simulink library "vlm_wing_lib"  (R2018b)
settings: Solver=VariableStepAuto  StartTime=0.0  StopTime=10.0  RelTol=1e-3
values from neighbouring files (symbols this model uses):
  wing = wingSetAeroState( wing, [0;0;0] )    [wingGet3dPolar.m]
undefined symbols (not defined in the file or in its folder): wing_struct, wing_struct_state, wing_struct_state_bus
libraries: $bdroot x6
settings Model: Creator=Ybeyer  LastModifiedBy=yannic
settings SFSimCC: SimUseLocalCustomCode=off
settings RTWCC: RTWUseLocalCustomCode=off
settings CodeAppCC: StateflowObjectComments=on

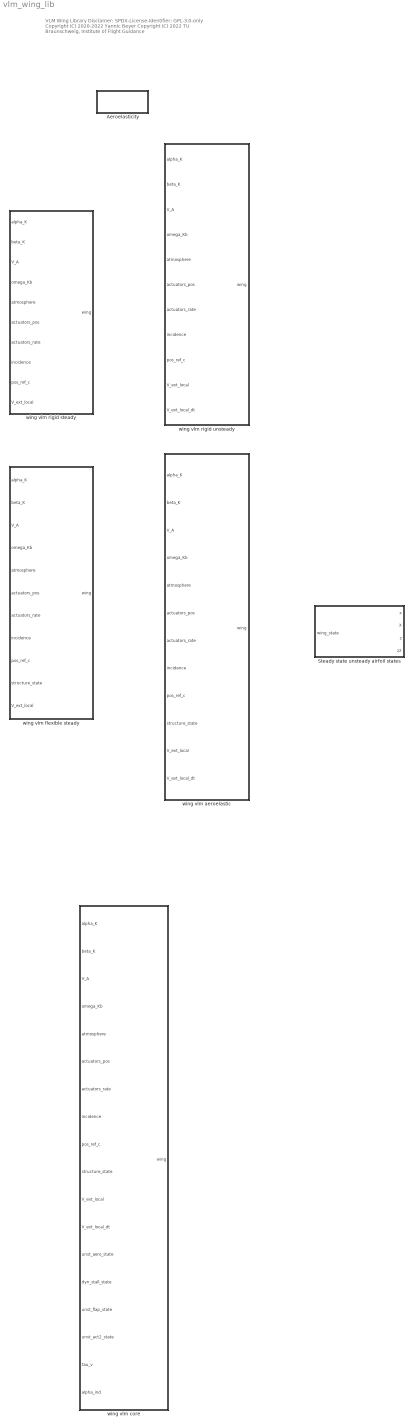
== system vlm_wing_lib ==
  note: VLM Wing Library
      |
      | Disclamer:
      | SPDX-License-Identifier: GPL-3.0-only
      |
      | Copyright (C) 2020-2022 Yannic Beyer
      | Copyright (C) 2022 TU Braunschweig, Institute of Flight Guidance
  Aeroelasticity : Subsystem
      settings: OpenFcn=aeroelasticity_lib
  Steady state unsteady airfoil states : Subsystem  mask{wing_airfoil=wing.airfoil, wing_config=wing.config}
      mask prompts: wing_airfoil "wing airfoil struct"; wing_config "wing config struct"
      mask DialogControl DescGroupVar Prompt: Compute steady state unsteady airfoil states
  wing vlm aeroelastic : Subsystem  mask{wing_struct=wing_struct, wing_state_bus=wing_struct_state, unst_aero_state_init=0, dyn_stall_state_init=0, unst_flap_state_init=0, unst_act2_state_init=0, tau_v_init=0, alpha_ind_init=0}
      mask prompts: wing_struct "Wing struct"; wing_state_bus "Wing state bus"; unst_aero_state_init "initial unst_aero_state"; dyn_stall_state_init "initial dyn_stall_state"; unst_flap_state_init "initial unst_flap_state"; unst_act2_state_init "initial unst_act2_state"; tau_v_init "initial tau_v"; alpha_ind_init "initial alpha_ind"
      mask Help: web('https://git.iff.ing.tu-bs.de/dev/flugmechanik/fdm/ladac/-/blob/feature/wing_improve_organization/aerodynamics/vlm_wing/README.md','-browser')
      mask DialogControl DescGroupVar Prompt: Wing with nonlinear vortex lattice method (aeroelastic)
      mask DialogControl DescTextVar Prompt: This block computes the aerodynamics of a wing based on the nonlinear vortex lattice method. It considers a flexible structure and unsteady aerodynamics.
      mask DialogControl Control12 Prompt: The inputs and outputs are described in the README:
      mask DialogControl Control5 Prompt: README
      mask DialogControl Control5 Callback: web('https://github.com/iff-gsc/LADAC/blob/main/aerodynamics/vlm_wing/README.md','-browser')
      mask DialogControl Control2 Prompt: To initialize a wing struct, please use the function wingCreate.
      mask DialogControl Control3 Prompt: The wing state bus can then be created by running wing_state_bus = struct2bus_(wing.state)
      mask DialogControl Container3 Prompt: Initial conditions
  wing vlm core : Subsystem  mask{wing_struct=wing_struct, wing_state_bus=wing_struct_state}
      mask prompts: wing_struct "Wing struct"; wing_state_bus "Wing state bus"
      mask Help: web('https://git.iff.ing.tu-bs.de/dev/flugmechanik/fdm/ladac/-/blob/feature/wing_improve_organization/aerodynamics/vlm_wing/README.md','-browser')
      mask DialogControl DescGroupVar Prompt: Wing with nonlinear vortex lattice method (aeroelastic)
      mask DialogControl DescTextVar Prompt: This block computes the aerodynamics of a wing based on the nonlinear vortex lattice method. It considers a flexible structure and unsteady aerodynamics.
      mask DialogControl Control12 Prompt: The inputs and outputs are described in the README:
      mask DialogControl Control5 Prompt: README
      mask DialogControl Control5 Callback: web('https://github.com/iff-gsc/LADAC/blob/main/aerodynamics/vlm_wing/README.md','-browser')
      mask DialogControl Control2 Prompt: To initialize a wing struct, please use the function wingCreate.
      mask DialogControl Control3 Prompt: The wing state bus can then be created by running wing_state_bus = struct2bus_(wing.state)
  wing vlm flexible steady : Subsystem  mask{wing_struct=wing_struct, wing_state_bus=wing_struct_state_bus, alpha_ind_init=0}
      mask prompts: wing_struct "Wing struct"; wing_state_bus "Wing state bus"; alpha_ind_init "initial alpha_ind"
      mask Help: web('https://git.iff.ing.tu-bs.de/dev/flugmechanik/fdm/ladac/-/blob/feature/wing_improve_organization/aerodynamics/vlm_wing/README.md','-browser')
      mask DialogControl DescGroupVar Prompt: Wing with nonlinear vortex lattice method (flexible steady)
      mask DialogControl DescTextVar Prompt: This block computes the aerodynamics of a wing based on the nonlinear vortex lattice method. It considers a flexible structure and steady aerodynamics.
      mask DialogControl Control2 Prompt: The inputs and outputs are described in the README:
      mask DialogControl Control5 Prompt: README
      mask DialogControl Control5 Callback: web('https://github.com/iff-gsc/LADAC/blob/main/aerodynamics/vlm_wing/README.md','-browser')
      mask DialogControl Control3 Prompt: To initialize a wing struct, please use the function wingCreate.
      mask DialogControl Control4 Prompt: The wing state bus can then be created by running wing_state_bus = struct2bus_(wing.state)
      mask DialogControl Container3 Prompt: Initial conditions
  wing vlm rigid steady : Subsystem  mask{wing_struct=wing_struct, wing_state_bus=wing_struct_state_bus, alpha_ind_init=0}
      mask prompts: wing_struct "Wing struct"; wing_state_bus "Wing state bus"; alpha_ind_init "initial alpha_ind"
      mask Help: web('https://git.iff.ing.tu-bs.de/dev/flugmechanik/fdm/ladac/-/blob/feature/wing_improve_organization/aerodynamics/vlm_wing/README.md','-browser')
      mask DialogControl DescGroupVar Prompt: Wing with nonlinear vortex lattice method (rigid steady)
      mask DialogControl DescTextVar Prompt: This block computes the aerodynamics of a wing based on the nonlinear vortex lattice method. It considers a rigid structure and steady aerodynamics.
      mask DialogControl Control2 Prompt: The inputs and outputs are described in the README:
      mask DialogControl Control5 Prompt: README
      mask DialogControl Control5 Callback: web('https://github.com/iff-gsc/LADAC/blob/main/aerodynamics/vlm_wing/README.md','-browser')
      mask DialogControl Control3 Prompt: To initialize a wing struct, please use the function wingCreate.
      mask DialogControl Control4 Prompt: The wing state bus can then be created by running wing_state_bus = struct2bus_(wing.state)
      mask DialogControl Container3 Prompt: Initial conditions
  wing vlm rigid unsteady : Subsystem  mask{wing_struct=wing_struct, wing_state_bus=wing_struct_state_bus, unst_aero_state_init=0, dyn_stall_state_init=0, unst_flap_state_init=0, unst_act2_state_init=0, tau_v_init=0, alpha_ind_init=0}
      mask prompts: wing_struct "Wing struct"; wing_state_bus "Wing state bus"; unst_aero_state_init "initial unst_aero_state"; dyn_stall_state_init "initial dyn_stall_state"; unst_flap_state_init "initial unst_flap_state"; unst_act2_state_init "initial unst_act2_state"; tau_v_init "initial tau_v"; alpha_ind_init "initial alpha_ind"
      mask Help: web('https://git.iff.ing.tu-bs.de/dev/flugmechanik/fdm/ladac/-/blob/feature/wing_improve_organization/aerodynamics/vlm_wing/README.md','-browser')
      mask DialogControl DescGroupVar Prompt: Wing with nonlinear vortex lattice method (flexible steady)
      mask DialogControl DescTextVar Prompt: This block computes the aerodynamics of a wing based on the nonlinear vortex lattice method. It considers a flexible structure and steady aerodynamics.
      mask DialogControl Control2 Prompt: The inputs and outputs are described in the README:
      mask DialogControl Control5 Prompt: README
      mask DialogControl Control5 Callback: web('https://github.com/iff-gsc/LADAC/blob/main/aerodynamics/vlm_wing/README.md','-browser')
      mask DialogControl Control3 Prompt: To initialize a wing struct, please use the function wingCreate.
      mask DialogControl Control4 Prompt: The wing state bus can then be created by running wing_state_bus = struct2bus_(wing.state)
      mask DialogControl Container3 Prompt: Initial conditions

== system vlm_wing_lib/Aeroelasticity ==

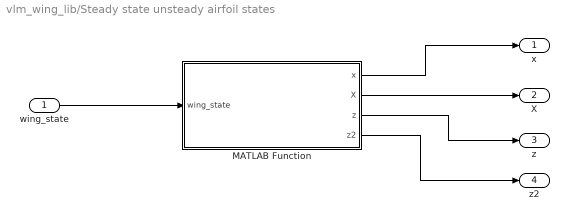
== system vlm_wing_lib/Steady state unsteady airfoil states ==
  wing_state : Inport
  MATLAB Function : MATLAB Function  TreatAsAtomicUnit=on
  x : Outport
  X : Outport  Port=2
  z : Outport  Port=3
  z2 : Outport  Port=4
  wires:
  MATLAB Function/4(z2) -> z2/1
  wing_state/1 -> MATLAB Function/1(wing_state)
  MATLAB Function/1(x) -> x/1
  MATLAB Function/2(X) -> X/1
  MATLAB Function/3(z) -> z/1

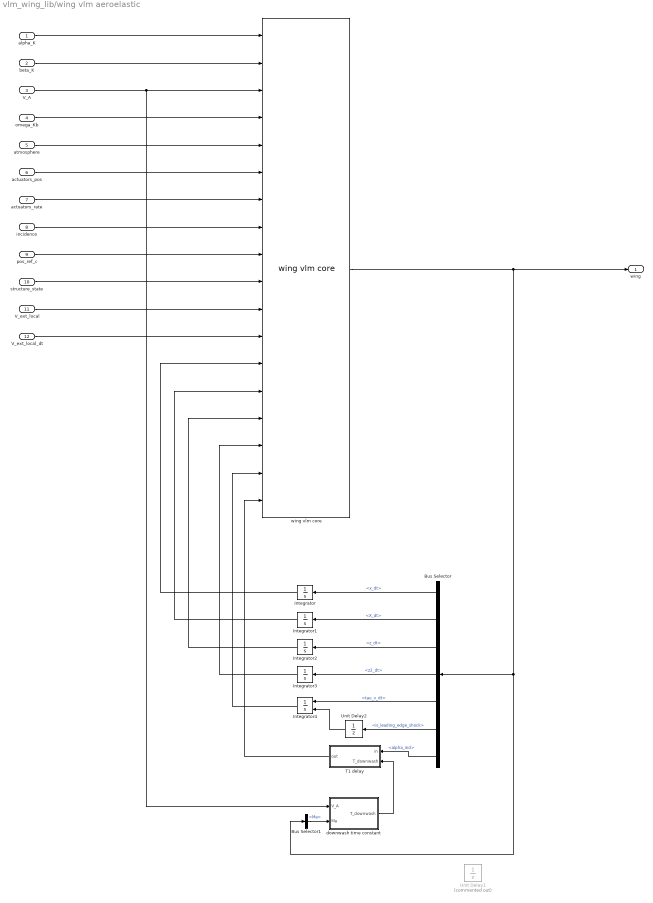
== system vlm_wing_lib/wing vlm aeroelastic ==
  alpha_K : Inport
  beta_K : Inport  Port=2
  V_A : Inport  Port=3
  omega_Kb : Inport  Port=4
  atmosphere : Inport  Port=5
  actuators_pos : Inport  Port=6
  actuators_rate : Inport  Port=7
  incidence : Inport  Port=8
  pos_ref_c : Inport  Port=9
  structure_state : Inport  Port=10
  V_ext_local : Inport  Port=11
  V_ext_local_dt : Inport  Port=12
  Bus Selector : BusSelector  OutputSignals=aero.unsteady.x_dt,aero.unsteady.X_dt,aero.unsteady.z_dt,aero.unsteady.z2_dt,aero.unsteady.tau_v_dt,aero.unsteady.is_leading_edge_shock,aero.circulation.alpha_ind
  Bus Selector1 : BusSelector  OutputSignals=aero.circulation.Ma
  Integrator : Integrator  InitialCondition=unst_aero_state_init
  Integrator1 : Integrator  InitialCondition=dyn_stall_state_init
  Integrator2 : Integrator  InitialCondition=unst_flap_state_init
  Integrator3 : Integrator  InitialCondition=unst_act2_state_init
  Integrator4 : Integrator  ExternalReset=falling  InitialCondition=tau_v_init
  T1 delay : Subsystem
  Unit Delay1 : UnitDelay  Commented=on  InitialCondition=alpha_ind_init  SampleTime=-1
  Unit Delay2 : UnitDelay  SampleTime=-1
  downwash time constant : Subsystem
  wing vlm core : $bdroot/wing vlm core  wing_struct=wing_struct  wing_state_bus=wing_state_bus
  wing : Outport
  wires:
  Integrator/1 -> wing vlm core/13
  Integrator1/1 -> wing vlm core/14
  Integrator2/1 -> wing vlm core/15
  Integrator3/1 -> wing vlm core/16
  Integrator4/1 -> wing vlm core/17
  T1 delay/1(out) -> wing vlm core/18
  Bus Selector/7 -> T1 delay/1(in)  "<alpha_ind>"
  Bus Selector/1 -> Integrator/1  "<x_dt>"
  Bus Selector/3 -> Integrator2/1  "<z_dt>"
  Bus Selector/4 -> Integrator3/1  "<z2_dt>"
  Bus Selector/5 -> Integrator4/1  "<tau_v_dt>"
  Bus Selector/6 -> Unit Delay2/1  "<is_leading_edge_shock>"
  Unit Delay2/1 -> Integrator4/2
  Bus Selector/2 -> Integrator1/1  "<X_dt>"
  alpha_K/1 -> wing vlm core/1
  beta_K/1 -> wing vlm core/2
  wing vlm core/1 -> Bus Selector1/1, Bus Selector/1, wing/1
  omega_Kb/1 -> wing vlm core/4
  atmosphere/1 -> wing vlm core/5
  actuators_pos/1 -> wing vlm core/6
  actuators_rate/1 -> wing vlm core/7
  incidence/1 -> wing vlm core/8
  pos_ref_c/1 -> wing vlm core/9
  structure_state/1 -> wing vlm core/10
  V_ext_local/1 -> wing vlm core/11
  V_ext_local_dt/1 -> wing vlm core/12
  downwash time constant/1(T_downwash) -> T1 delay/2(T_downwash)
  Bus Selector1/1 -> downwash time constant/2(Ma)  "<Ma>"
  V_A/1 -> downwash time constant/1(V_A), wing vlm core/3

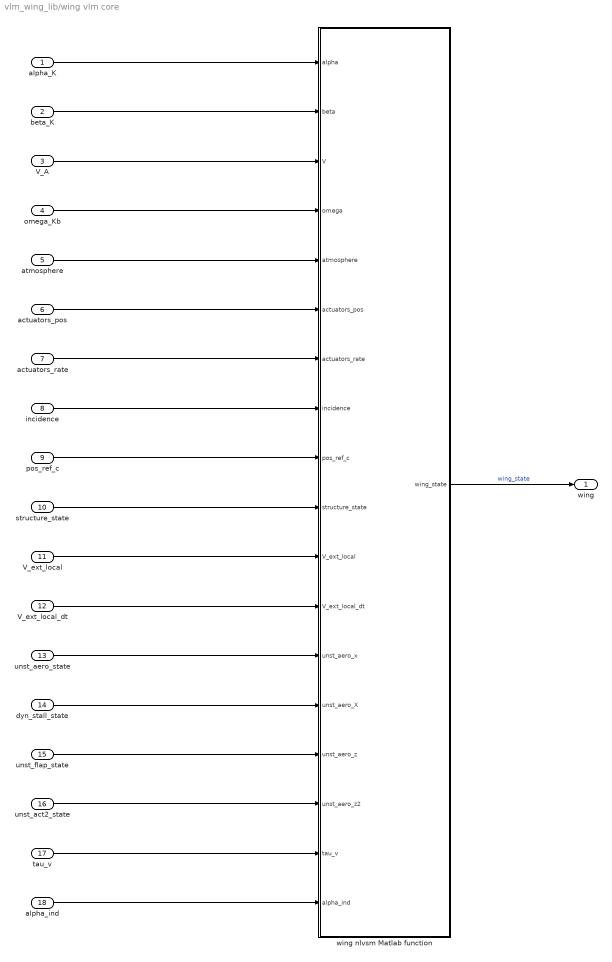
== system vlm_wing_lib/wing vlm core ==
  alpha_K : Inport
  beta_K : Inport  Port=2
  V_A : Inport  Port=3
  omega_Kb : Inport  Port=4
  atmosphere : Inport  Port=5
  actuators_pos : Inport  Port=6
  actuators_rate : Inport  Port=7
  incidence : Inport  Port=8
  pos_ref_c : Inport  Port=9
  structure_state : Inport  Port=10
  V_ext_local : Inport  Port=11
  V_ext_local_dt : Inport  Port=12
  unst_aero_state : Inport  Port=13
  dyn_stall_state : Inport  Port=14
  unst_flap_state : Inport  Port=15
  unst_act2_state : Inport  Port=16
  tau_v : Inport  Port=17
  alpha_ind : Inport  Port=18
  wing nlvsm Matlab function : MATLAB Function  TreatAsAtomicUnit=on
  wing : Outport
  wires:
  unst_aero_state/1 -> wing nlvsm Matlab function/13(unst_aero_x)
  structure_state/1 -> wing nlvsm Matlab function/10(structure_state)
  wing nlvsm Matlab function/1(wing_state) -> wing/1  "wing_state"
  incidence/1 -> wing nlvsm Matlab function/8(incidence)
  V_A/1 -> wing nlvsm Matlab function/3(V)
  alpha_K/1 -> wing nlvsm Matlab function/1(alpha)
  omega_Kb/1 -> wing nlvsm Matlab function/4(omega)
  pos_ref_c/1 -> wing nlvsm Matlab function/9(pos_ref_c)
  atmosphere/1 -> wing nlvsm Matlab function/5(atmosphere)
  beta_K/1 -> wing nlvsm Matlab function/2(beta)
  actuators_rate/1 -> wing nlvsm Matlab function/7(actuators_rate)
  actuators_pos/1 -> wing nlvsm Matlab function/6(actuators_pos)
  dyn_stall_state/1 -> wing nlvsm Matlab function/14(unst_aero_X)
  unst_flap_state/1 -> wing nlvsm Matlab function/15(unst_aero_z)
  unst_act2_state/1 -> wing nlvsm Matlab function/16(unst_aero_z2)
  V_ext_local/1 -> wing nlvsm Matlab function/11(V_ext_local)
  V_ext_local_dt/1 -> wing nlvsm Matlab function/12(V_ext_local_dt)
  tau_v/1 -> wing nlvsm Matlab function/17(tau_v)
  alpha_ind/1 -> wing nlvsm Matlab function/18(alpha_ind)

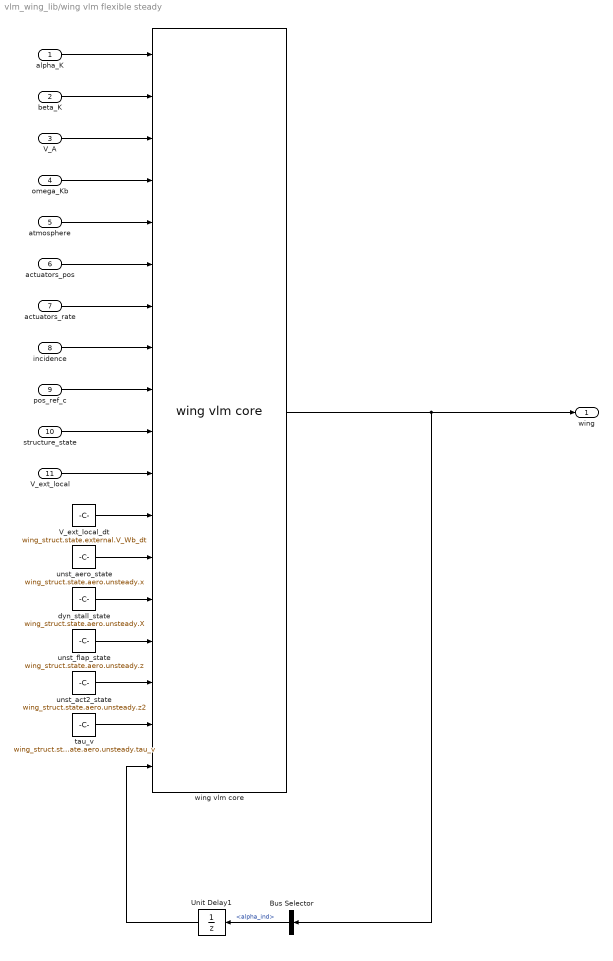
== system vlm_wing_lib/wing vlm flexible steady ==
  alpha_K : Inport
  beta_K : Inport  Port=2
  V_A : Inport  Port=3
  omega_Kb : Inport  Port=4
  atmosphere : Inport  Port=5
  actuators_pos : Inport  Port=6
  actuators_rate : Inport  Port=7
  incidence : Inport  Port=8
  pos_ref_c : Inport  Port=9
  structure_state : Inport  Port=10
  V_ext_local : Inport  Port=11
  Bus Selector : BusSelector  OutputSignals=aero.circulation.alpha_ind
  Unit Delay1 : UnitDelay  InitialCondition=alpha_ind_init  SampleTime=-1
  V_ext_local_dt : Constant  Value=wing_struct.state.external.V_Wb_dt
  dyn_stall_state : Constant  Value=wing_struct.state.aero.unsteady.X
  tau_v : Constant  Value=wing_struct.state.aero.unsteady.tau_v
  unst_act2_state : Constant  Value=wing_struct.state.aero.unsteady.z2
  unst_aero_state : Constant  Value=wing_struct.state.aero.unsteady.x
  unst_flap_state : Constant  Value=wing_struct.state.aero.unsteady.z
  wing vlm core : $bdroot/wing vlm core  wing_struct=wing_struct  wing_state_bus=wing_state_bus
  wing : Outport
  wires:
  pos_ref_c/1 -> wing vlm core/9
  incidence/1 -> wing vlm core/8
  actuators_rate/1 -> wing vlm core/7
  actuators_pos/1 -> wing vlm core/6
  atmosphere/1 -> wing vlm core/5
  omega_Kb/1 -> wing vlm core/4
  V_A/1 -> wing vlm core/3
  beta_K/1 -> wing vlm core/2
  alpha_K/1 -> wing vlm core/1
  structure_state/1 -> wing vlm core/10
  V_ext_local/1 -> wing vlm core/11
  V_ext_local_dt/1 -> wing vlm core/12
  unst_aero_state/1 -> wing vlm core/13
  dyn_stall_state/1 -> wing vlm core/14
  unst_flap_state/1 -> wing vlm core/15
  unst_act2_state/1 -> wing vlm core/16
  tau_v/1 -> wing vlm core/17
  wing vlm core/1 -> Bus Selector/1, wing/1
  Unit Delay1/1 -> wing vlm core/18
  Bus Selector/1 -> Unit Delay1/1  "<alpha_ind>"

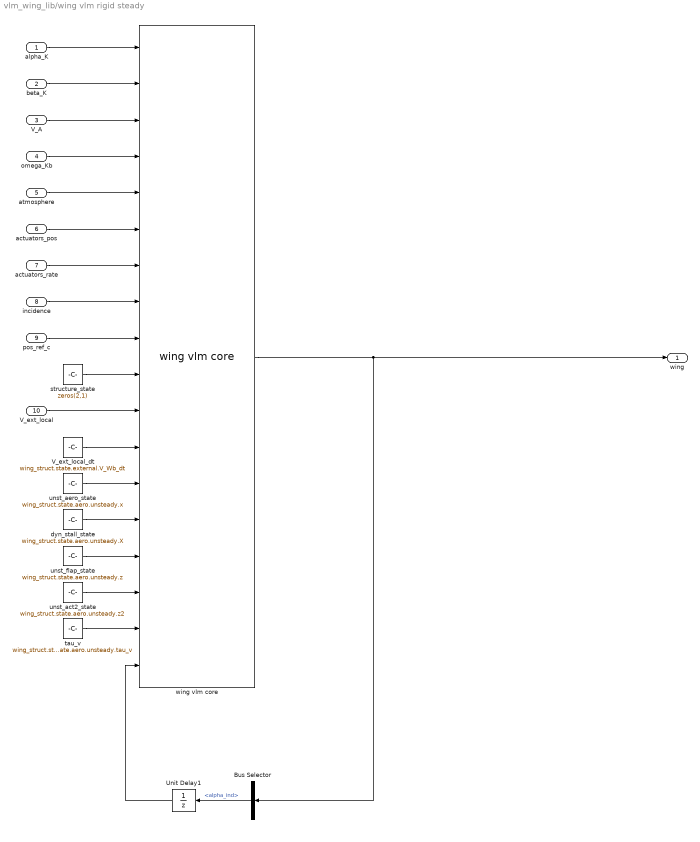
== system vlm_wing_lib/wing vlm rigid steady ==
  alpha_K : Inport
  beta_K : Inport  Port=2
  V_A : Inport  Port=3
  omega_Kb : Inport  Port=4
  atmosphere : Inport  Port=5
  actuators_pos : Inport  Port=6
  actuators_rate : Inport  Port=7
  incidence : Inport  Port=8
  pos_ref_c : Inport  Port=9
  V_ext_local : Inport  Port=10
  Bus Selector : BusSelector  OutputSignals=aero.circulation.alpha_ind
  Unit Delay1 : UnitDelay  InitialCondition=alpha_ind_init  SampleTime=-1
  V_ext_local_dt : Constant  Value=wing_struct.state.external.V_Wb_dt
  dyn_stall_state : Constant  Value=wing_struct.state.aero.unsteady.X
  structure_state : Constant  Value=zeros(2,1)  VectorParams1D=off
  tau_v : Constant  Value=wing_struct.state.aero.unsteady.tau_v
  unst_act2_state : Constant  Value=wing_struct.state.aero.unsteady.z2
  unst_aero_state : Constant  Value=wing_struct.state.aero.unsteady.x
  unst_flap_state : Constant  Value=wing_struct.state.aero.unsteady.z
  wing vlm core : $bdroot/wing vlm core  wing_struct=wing_struct  wing_state_bus=wing_state_bus
  wing : Outport
  wires:
  V_ext_local/1 -> wing vlm core/11
  V_ext_local_dt/1 -> wing vlm core/12
  unst_aero_state/1 -> wing vlm core/13
  dyn_stall_state/1 -> wing vlm core/14
  unst_flap_state/1 -> wing vlm core/15
  unst_act2_state/1 -> wing vlm core/16
  tau_v/1 -> wing vlm core/17
  Unit Delay1/1 -> wing vlm core/18
  structure_state/1 -> wing vlm core/10
  pos_ref_c/1 -> wing vlm core/9
  incidence/1 -> wing vlm core/8
  actuators_rate/1 -> wing vlm core/7
  actuators_pos/1 -> wing vlm core/6
  atmosphere/1 -> wing vlm core/5
  omega_Kb/1 -> wing vlm core/4
  V_A/1 -> wing vlm core/3
  beta_K/1 -> wing vlm core/2
  alpha_K/1 -> wing vlm core/1
  Bus Selector/1 -> Unit Delay1/1  "<alpha_ind>"
  wing vlm core/1 -> Bus Selector/1, wing/1

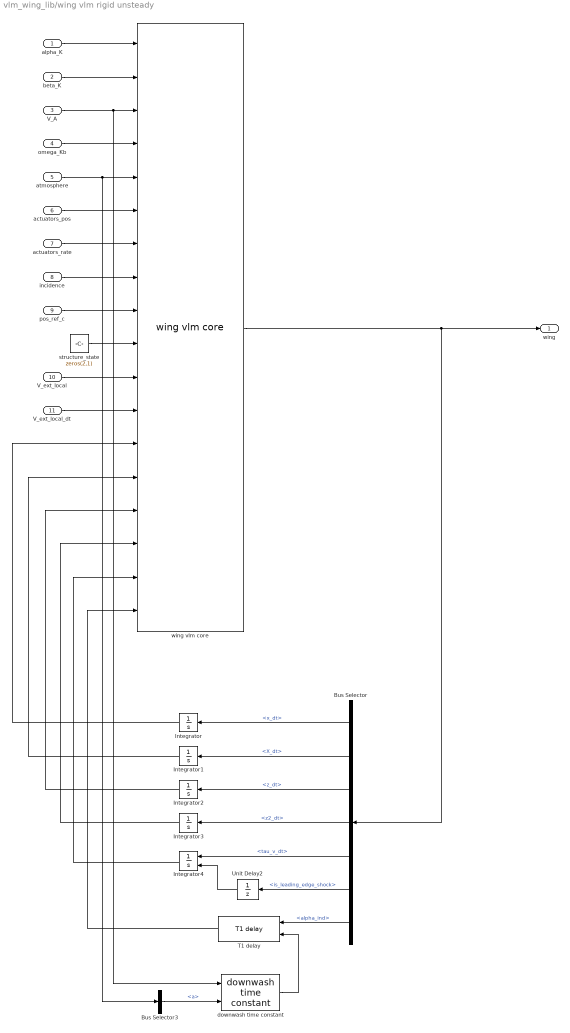
== system vlm_wing_lib/wing vlm rigid unsteady ==
  alpha_K : Inport
  beta_K : Inport  Port=2
  V_A : Inport  Port=3
  omega_Kb : Inport  Port=4
  atmosphere : Inport  Port=5
  actuators_pos : Inport  Port=6
  actuators_rate : Inport  Port=7
  incidence : Inport  Port=8
  pos_ref_c : Inport  Port=9
  V_ext_local : Inport  Port=10
  V_ext_local_dt : Inport  Port=11
  Bus Selector : BusSelector  OutputSignals=aero.unsteady.x_dt,aero.unsteady.X_dt,aero.unsteady.z_dt,aero.unsteady.z2_dt,aero.unsteady.tau_v_dt,aero.unsteady.is_leading_edge_shock,aero.circulation.alpha_ind
  Bus Selector3 : BusSelector  OutputSignals=a
  Integrator : Integrator  InitialCondition=unst_aero_state_init
  Integrator1 : Integrator  InitialCondition=dyn_stall_state_init
  Integrator2 : Integrator  InitialCondition=unst_flap_state_init
  Integrator3 : Integrator  InitialCondition=unst_act2_state_init
  Integrator4 : Integrator  ExternalReset=falling  InitialCondition=tau_v_init
  T1 delay : $bdroot/wing vlm aeroelastic/T1 delay  SystemSampleTime=-1
  Unit Delay2 : UnitDelay  SampleTime=-1
  downwash time constant : $bdroot/wing vlm aeroelastic/downwash time constant  SystemSampleTime=-1
  structure_state : Constant  Value=zeros(2,1)  VectorParams1D=off
  wing vlm core : $bdroot/wing vlm core  wing_struct=wing_struct  wing_state_bus=wing_state_bus
  wing : Outport
  wires:
  pos_ref_c/1 -> wing vlm core/9
  incidence/1 -> wing vlm core/8
  actuators_rate/1 -> wing vlm core/7
  actuators_pos/1 -> wing vlm core/6
  omega_Kb/1 -> wing vlm core/4
  beta_K/1 -> wing vlm core/2
  alpha_K/1 -> wing vlm core/1
  structure_state/1 -> wing vlm core/10
  V_ext_local/1 -> wing vlm core/11
  V_ext_local_dt/1 -> wing vlm core/12
  Bus Selector/4 -> Integrator3/1  "<z2_dt>"
  Bus Selector/1 -> Integrator/1  "<x_dt>"
  T1 delay/1 -> wing vlm core/18
  Bus Selector/2 -> Integrator1/1  "<X_dt>"
  Bus Selector/3 -> Integrator2/1  "<z_dt>"
  Bus Selector/5 -> Integrator4/1  "<tau_v_dt>"
  Bus Selector/7 -> T1 delay/1  "<alpha_ind>"
  Bus Selector/6 -> Unit Delay2/1  "<is_leading_edge_shock>"
  Unit Delay2/1 -> Integrator4/2
  Integrator4/1 -> wing vlm core/17
  Integrator3/1 -> wing vlm core/16
  Integrator1/1 -> wing vlm core/14
  Integrator2/1 -> wing vlm core/15
  wing vlm core/1 -> Bus Selector/1, wing/1
  Integrator/1 -> wing vlm core/13
  atmosphere/1 -> wing vlm core/5, Bus Selector3/1
  Bus Selector3/1 -> downwash time constant/2  "<a>"
  V_A/1 -> downwash time constant/1, wing vlm core/3
  downwash time constant/1 -> T1 delay/2

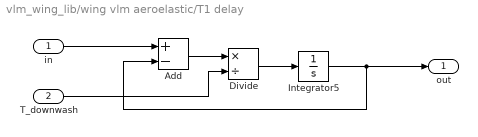
== system vlm_wing_lib/wing vlm aeroelastic/T1 delay ==
  in : Inport
  T_downwash : Inport  Port=2
  Add : Sum  Inputs=+-
  Divide : Product  Inputs=*/
  Integrator5 : Integrator  InitialCondition=alpha_ind_init
  out : Outport
  wires:
  Divide/1 -> Integrator5/1
  Add/1 -> Divide/1
  Integrator5/1 -> out/1, Add/2
  in/1 -> Add/1
  T_downwash/1 -> Divide/2

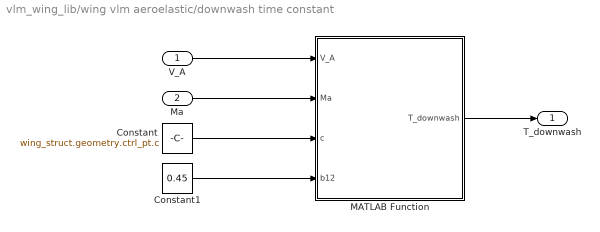
== system vlm_wing_lib/wing vlm aeroelastic/downwash time constant ==
  V_A : Inport
  Ma : Inport  Port=2
  Constant : Constant  Value=wing_struct.geometry.ctrl_pt.c  VectorParams1D=off
  Constant1 : Constant  Value=0.45
  MATLAB Function : MATLAB Function  TreatAsAtomicUnit=on
  T_downwash : Outport
  wires:
  Constant/1 -> MATLAB Function/3(c)
  Constant1/1 -> MATLAB Function/4(b12)
  V_A/1 -> MATLAB Function/1(V_A)
  Ma/1 -> MATLAB Function/2(Ma)
  MATLAB Function/1(T_downwash) -> T_downwash/1

== matlab function vlm_wing_lib/wing vlm core/wing nlvsm Matlab function ==
  data: wing_struct parameter; alpha input; wing_state output wing_state_bus; beta input; V input; omega input; atmosphere input; actuators_pos input; actuators_rate input; incidence input; pos_ref_c input; structure_state input; V_ext_local input; V_ext_local_dt input; unst_aero_x input; unst_aero_X input; unst_aero_z input; unst_aero_z2 input; tau_v input; alpha_ind input
function wing_state  = fcn( wing_struct, alpha, beta, V, omega, ...
    atmosphere, actuators_pos, actuators_rate, ...
    incidence, pos_ref_c, structure_state, ...
    V_ext_local, V_ext_local_dt, ...
    unst_aero_x, unst_aero_X, unst_aero_z, unst_aero_z2, tau_v, ...
    alpha_ind ) %#codegen

%% incidence
wing_struct.state.geometry.ctrl_pt.local_incidence = wing_struct.geometry.ctrl_pt.local_incidence + incidence;

%% compute wing state
wing_struct = wingSetState( wing_struct, alpha, beta, V, omega, ...
    actuators_pos, actuators_rate, pos_ref_c, 'atmosphere', atmosphere, ...
    'V_Wb', V_ext_local, 'V_Wb_dt', V_ext_local_dt, ...
    'structure_pos', structure_state(1:end/2), 'structure_vel', structure_state(end/2+1:end), ...
    'unst_airfoil_state', unst_aero_x, 'dyn_stall_state', unst_aero_X, ...
    'unst_flap_state', unst_aero_z, 'unst_act2_state', unst_aero_z2, ...
    'tau_v', tau_v, 'alpha_ind', alpha_ind );

wing_state      = wing_struct.state;

end

== matlab function vlm_wing_lib/wing vlm aeroelastic/downwash time constant/MATLAB Function ==
  data: V_A input; T_downwash output; Ma input; c input; b12 input
function T_downwash = fcn(V_A, Ma, c,  b12)
% This time constant is similar to the time constant for the 2D airfoil.
% Validation will show if this assuption is correct but it should not be
% too wrong.

Ma(Ma>0.95) = 0.95;

beta_Ma = sqrt( 1 - Ma.^2 );

T_downwash = 1 ./ ( (2*V_A./c).*beta_Ma.^2*b12 );

end

== matlab function vlm_wing_lib/Steady state unsteady airfoil states/MATLAB Function ==
  data: wing_state input; x output; X output; z output; z2 output; wing_airfoil parameter; wing_config parameter
function [x,X,z,z2] = wingStateGetUnstAeroTrimOp( wing_state, wing_airfoil, wing_config)

[x,X,z,z2] = wingStateGetUnstAeroTrimOp( wing_state, wing_airfoil, wing_config );

end
